simulink model "Hybrid_OpAmp_Differential"
settings: Solver=ode23t  StopTime=0.002  RelTol=1e-5  AbsTol=1e-6
settings Model: Creator=Senior Analog IC & SET Device Design Engineer  LastModifiedBy=Antigravity MATLAB Automation

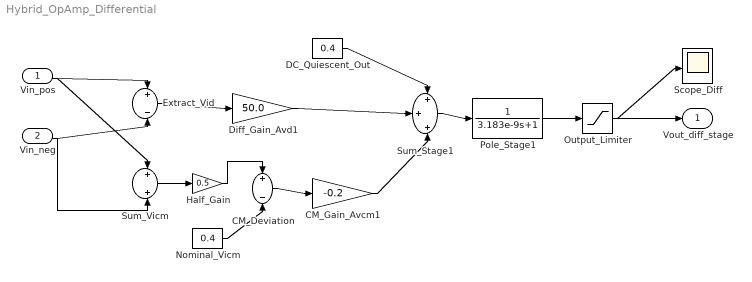
== system Hybrid_OpAmp_Differential ==
  Vin_pos : Inport  Port=1
  Vin_neg : Inport  Port=2
  Extract_Vid : Sum  Inputs=+-
  Sum_Vicm : Sum  Inputs=++
  Half_Gain : Gain  Gain=0.5
  Diff_Gain_Avd1 : Gain  Gain=50.0
  Nominal_Vicm : Constant  Value=0.4
  CM_Deviation : Sum  Inputs=+-
  CM_Gain_Avcm1 : Gain  Gain=-0.2
  DC_Quiescent_Out : Constant  Value=0.4
  Sum_Stage1 : Sum  Inputs=+++
  Pole_Stage1 : TransferFcn  Numerator=[1]  Denominator=[3.183e-9 1]
  Output_Limiter : Saturate  UpperLimit=0.75  LowerLimit=0.05
  Vout_diff_stage : Outport  Port=1
  Scope_Diff : Scope
  wires:
  Vin_pos/1 -> Extract_Vid/1
  Vin_neg/1 -> Extract_Vid/2
  Vin_pos/1 -> Sum_Vicm/1
  Vin_neg/1 -> Sum_Vicm/2
  Sum_Vicm/1 -> Half_Gain/1
  Extract_Vid/1 -> Diff_Gain_Avd1/1
  Half_Gain/1 -> CM_Deviation/1
  Nominal_Vicm/1 -> CM_Deviation/2
  CM_Deviation/1 -> CM_Gain_Avcm1/1
  DC_Quiescent_Out/1 -> Sum_Stage1/1
  Diff_Gain_Avd1/1 -> Sum_Stage1/2
  CM_Gain_Avcm1/1 -> Sum_Stage1/3
  Sum_Stage1/1 -> Pole_Stage1/1
  Pole_Stage1/1 -> Output_Limiter/1
  Output_Limiter/1 -> Vout_diff_stage/1
  Output_Limiter/1 -> Scope_Diff/1
